simulink model "Bossi_Emanuele_EE460S3D_R99"  (R2025a)
settings: Solver=FixedStepDiscrete  StartTime=0.0  StopTime=120  FixedStep=dt0  RelTol=1e-3  EnableMultiTasking=on
PostLoadFcn:
  | %Set the size for the model
  | set_param(gcs,'Location',[10 10 1270 970])
  | %Set the zoom factor for the model
  | set_param(gcs,'ZoomFactor','100')
InitFcn:
  | tic
  | Bossi_Emanuele_EE460_Final
  | INIT_S3D_01
StartFcn:
  | tend0=toc;
  | tic;
StopFcn:
  | tend=toc;
  | disp(['Simulation time = ' num2str(tout(end)) ' sec'])
  | disp(['Real time = ' num2str(tend) ' sec'])
  | title('DONE')
  | SCORE=round((max(0,120-tout(end)-tend0))*4+10*(40-FuelBurned)+sum(100*double(PDONE)-100*double(PDONE<.5)));
  | PlotS3D(PlotInput);
  | text(15,22,['S: ' num2str(SCORE)]);
  | % Reset color scheme back to normal defaults
  | figure()
  | blkwhitebg('w');
  | close
values from neighbouring files (symbols this model uses):
  A_obs = [ 0  1  0  0  0  0 ... (first row only)    [Bossi_Emanuele_EE460_Final.m]
  B_obs = [ 0     0     0 ... (first row only)    [Bossi_Emanuele_EE460_Final.m]
  C_obs = [ 1 0 0 0 0 0 ... (first row only)    [Bossi_Emanuele_EE460_Final.m]
  d2r = pi/180    (= 0.0174532925199)    [INIT_S3D_01.m]
  D_obs = [ 0     0     0 ... (first row only)    [Bossi_Emanuele_EE460_Final.m]
  dt = 0.01    [INIT_S3D_01.m]
  dt0 = 0.001    [INIT_S3D_01.m]
  fr = 100    [INIT_S3D_01.m]
  G = [1,  1, -1, -1,  0,  0,  0,  0 ... (first row only)    [Bossi_Emanuele_EE460_Final.m]
  G_obs = eye(6)    [Bossi_Emanuele_EE460_Final.m]
  HM_S = 250    [INIT_S3D_01.m]
  HM_U = 500    [INIT_S3D_01.m]
  J = Jbase+JC0+JF+M*(Xcg^2+Ycg^2)    [INIT_S3D_01.m]
  Jbase = JC1+4*Ja+2*Ma*da^2+2*Ma*db^2    [INIT_S3D_01.m]
  JC0 = MC0/2    (= 10.2101761242)    [INIT_S3D_01.m]
  Kdtheta = 2 * zeta_th * wn_th * J_eff    [Bossi_Emanuele_EE460_Final.m]
  Kdtheta_fail = 2 * zeta_th_fail * wn_th_fail * J_eff    [Bossi_Emanuele_EE460_Final.m]
  Kdx = 2 * zeta_xy * wn_xy * M_eff    [Bossi_Emanuele_EE460_Final.m]
  Kdx_fail = 2 * zeta_xy_fail * wn_xy_fail * M_eff    [Bossi_Emanuele_EE460_Final.m]
  Kdy = 2 * zeta_xy * wn_xy * M_eff    [Bossi_Emanuele_EE460_Final.m]
  Kdy_fail = 2 * zeta_xy_fail * wn_xy_fail * M_eff    [Bossi_Emanuele_EE460_Final.m]
  Kptheta = J_eff * wn_th^2    [Bossi_Emanuele_EE460_Final.m]
  Kptheta_fail = J_eff * wn_th_fail^2    [Bossi_Emanuele_EE460_Final.m]
  Kpx = M_eff * wn_xy^2    [Bossi_Emanuele_EE460_Final.m]
  Kpx_fail = M_eff * wn_xy_fail^2    [Bossi_Emanuele_EE460_Final.m]
  Kpy = M_eff * wn_xy^2    [Bossi_Emanuele_EE460_Final.m]
  Kpy_fail = M_eff * wn_xy_fail^2    [Bossi_Emanuele_EE460_Final.m]
  L13 = sqrt(10)    [INIT_S3D_01.m]
  L24 = sqrt(6.25)    [INIT_S3D_01.m]
  LVL = LVL12    [INIT_S3D_01.m]
  M = MC+M1+M2+M3+M4+4*Ma    [INIT_S3D_01.m]
  M1 = LVL.M1    [INIT_S3D_01.m]
  M2 = LVL.M2    [INIT_S3D_01.m]
  M3 = LVL.M3    [INIT_S3D_01.m]
  M4 = LVL.M4    [INIT_S3D_01.m]
  max_qddot = [max_qddot_x; max_qddot_y; max_qddot_theta]    [Bossi_Emanuele_EE460_Final.m]
  mdti = (1/300)    (= 0.00333333333333)    [INIT_S3D_01.m]
  P = [1  1 -1 -1  0  0  0  0 ... (first row only)    [Bossi_Emanuele_EE460_Final.m]
  Pdata = [LVL.P1 LVL.P2 LVL.P3 LVL.P4]    [INIT_S3D_01.m]    (also in PlotS3D.m = R*[xt1;yt1+[0 3*tt*TV(idx-13)*TSIG(idx-13) 0]])
  PTvec = [Pdata(:,1);Pdata(:,2);Pdata(:,3);Pdata(:,4) ... (first row only)    [INIT_S3D_01.m]
  Q_obs = eye(6)    [Bossi_Emanuele_EE460_Final.m]
  r2d = 180/pi    (= 57.2957795131)    [INIT_S3D_01.m]
  r_bang = 0.5    [Bossi_Emanuele_EE460_Final.m]
  Sconfig = 1    [Bossi_Emanuele_EE460_Final.m]
  SLIM = [-100 100 ... (first row only)    [INIT_S3D_01.m]
  SQ = [.005 .01 .004 .005 .01 .004 .02 .01 .4]'    [INIT_S3D_01.m]
  SSF = 1./SQ    [INIT_S3D_01.m]
  tau = 0.5    [Bossi_Emanuele_EE460_Final.m]
  TOLdata = [LVL.P1tol LVL.P2tol LVL.P3tol LVL.P4tol]    [INIT_S3D_01.m]
  ULIM = [[Umin Umax];0 0;0 0]    [INIT_S3D_01.m]
undefined symbols (not defined in the file or in its folder): den_lp, den_lp2, DiscIntNeverNeededParam, dt1_bang_3, dt2_bang_3, dtc_bang_3, num_lp, num_lp2, q0_1
libraries: simulink x87, matrix_library x4, sl3dlib x1, aerolibutil x1, aerolibanimutils x1
(part 2 of 8)

== system Bossi_Emanuele_EE460S3D_R99/ControlLaw/ControlAllocation/A ==
  Y_IN : Inport
  Bus Creator : BusCreator  Inputs=2
  Bus Selector : BusSelector  OutputSignals=PT,Minv
  Constant1 : Constant  Value=P
  Constant2 : Constant  Value=P
  Gain : Gain  Gain=2
  Invert 3x3 Matrix : aerolibutil/Invert  3x3 Matrix
  MatrixMultiply{,1..3} (4 alike) : Product  Multiplication=Matrix(*)
  Transpose : Math  Operator=transpose
  WTI : Subsystem
  Out1 : Outport
  wires:
  Y_IN/1 -> WTI/1(Y_IN)
  WTI/1(Out1) -> MatrixMultiply3/1, MatrixMultiply1/2
  Constant1/1 -> MatrixMultiply1/1
  MatrixMultiply1/1 -> MatrixMultiply2/1
  Constant2/1 -> Transpose/1
  Transpose/1 -> Bus Creator/2, MatrixMultiply2/2  "PT"
  MatrixMultiply2/1 -> Invert 3x3 Matrix/1  "M"
  MatrixMultiply/1 -> MatrixMultiply3/2
  MatrixMultiply3/1 -> Gain/1  "A"
  Gain/1 -> Out1/1  "2A"
  Invert 3x3 Matrix/1 -> Bus Creator/1  "Minv"
  Bus Creator/1 -> Bus Selector/1
  Bus Selector/1 -> MatrixMultiply/1  "<PT>"
  Bus Selector/2 -> MatrixMultiply/2  "<Minv>"

== system Bossi_Emanuele_EE460S3D_R99/ControlLaw/ControlAllocation/BodyAxisModeling ==
  uP_cmd : Inport  PortDimensions=3
  theta_rad : Inport  Port=2
  Bus Creator : BusCreator  Inputs=5
  Bus Creator1 : BusCreator  Inputs=4
  Bus Selector : BusSelector  OutputSignals=Fx_N,c,c,Fy_N,Fy_N,s,Fx_N,s,Mz_Nm
  Bus Selector1 : BusSelector  OutputSignals=cFx,sFy,cFy,sFx
  Demux1 : Demux  Outputs=3
  FxB_sum1 : Sum  Inputs=|++
  Mux2 : Mux  Inputs=3
  Sum1 : Sum
  cFx1 : Product
  cFy1 : Product
  cos_theta1 : Trigonometry  Operator=cos
  neg2 : Gain  Gain=-1
  sFx1 : Product
  sFy1 : Product
  sin_theta1 : Trigonometry
  Out1 : Outport
  wires:
  uP_cmd/1 -> Demux1/1  "uP_cmd"
  cos_theta1/1 -> Bus Creator/1  "c"
  sin_theta1/1 -> Bus Creator/2  "s"
  Demux1/1 -> Bus Creator/3  "Fx_N"
  Demux1/2 -> Bus Creator/4  "Fy_N"
  Demux1/3 -> Bus Creator/5  "Mz_Nm"
  Bus Creator/1 -> Bus Selector/1
  Bus Selector/1 -> cFx1/1  "<Fx_N>"
  Bus Selector/2 -> cFx1/2  "<c>"
  Bus Selector/3 -> cFy1/1  "<c>"
  Bus Selector/4 -> cFy1/2  "<Fy_N>"
  Bus Selector/5 -> sFy1/1  "<Fy_N>"
  Bus Selector/6 -> sFy1/2  "<s>"
  Bus Selector/7 -> sFx1/1  "<Fx_N>"
  Bus Selector/8 -> sFx1/2  "<s>"
  cFx1/1 -> Bus Creator1/1  "cFx"
  cFy1/1 -> Bus Creator1/2  "cFy"
  sFy1/1 -> Bus Creator1/3  "sFy"
  sFx1/1 -> Bus Creator1/4  "sFx"
  Bus Creator1/1 -> Bus Selector1/1
  neg2/1 -> Sum1/2
  Bus Selector/9 -> Mux2/3  "<Mz_Nm>"
  Bus Selector1/1 -> FxB_sum1/1  "<cFx>"
  Bus Selector1/2 -> FxB_sum1/2  "<sFy>"
  FxB_sum1/1 -> Mux2/1  "FxB_pos"
  Bus Selector1/3 -> Sum1/1  "<cFy>"
  Bus Selector1/4 -> neg2/1  "<sFx>"
  Sum1/1 -> Mux2/2  "FyB_pos"
  theta_rad/1 -> sin_theta1/1, cos_theta1/1
  Mux2/1 -> Out1/1  "uP_body"

== system Bossi_Emanuele_EE460S3D_R99/ControlLaw/ControlAllocation/R_theta ==
  In2 : Inport
  Bus Creator : BusCreator  Inputs=5
  Bus Selector : BusSelector  OutputSignals=c,minus_s,z0,s,c,z0,z0,z0,z1
  Constant : Constant  Value=0  SampleTime=dt
  Constant1 : Constant  SampleTime=dt
  Cos : Trigonometry  Operator=cos
  Gain : Gain  Gain=-1
  Matrix Concatenate : Concatenate  NumInputs=3  Mode=Multidimensional array
  Mux : Mux  Inputs=3
  Mux1 : Mux  Inputs=3
  Mux2 : Mux  Inputs=3
  Reshape : Reshape  OutputDimensionality=Customize  OutputDimensions=[1,3]
  Reshape1 : Reshape  OutputDimensionality=Customize  OutputDimensions=[1,3]
  Reshape2 : Reshape  OutputDimensionality=Customize  OutputDimensions=[1,3]
  Sin : Trigonometry
  Out1 : Outport
  wires:
  In2/1 -> Sin/1, Cos/1
  Sin/1 -> Gain/1, Bus Creator/4  "s"
  Cos/1 -> Bus Creator/3  "c"
  Gain/1 -> Bus Creator/5  "minus_s"
  Constant/1 -> Bus Creator/1  "z0"
  Constant1/1 -> Bus Creator/2  "z1"
  Bus Creator/1 -> Bus Selector/1
  Matrix Concatenate/1 -> Out1/1  "R"
  Bus Selector/1 -> Mux/1  "<c>"
  Bus Selector/2 -> Mux/2  "<minus_s>"
  Bus Selector/3 -> Mux/3  "<z0>"
  Bus Selector/4 -> Mux1/1  "<s>"
  Bus Selector/5 -> Mux1/2  "<c>"
  Bus Selector/6 -> Mux1/3  "<z0>"
  Bus Selector/7 -> Mux2/1  "<z0>"
  Bus Selector/8 -> Mux2/2  "<z0>"
  Bus Selector/9 -> Mux2/3  "<z1>"
  Mux/1 -> Reshape/1
  Reshape/1 -> Matrix Concatenate/1
  Reshape1/1 -> Matrix Concatenate/2
  Mux1/1 -> Reshape1/1
  Mux2/1 -> Reshape2/1
  Reshape2/1 -> Matrix Concatenate/3

== system Bossi_Emanuele_EE460S3D_R99/ControlLaw/ControlAllocation/ThrusterFailure ==
  Y_IN : Inport
  Bus Creator1 : BusCreator  Inputs=8
  Bus Creator2 : BusCreator  Inputs=8
  Bus Selector3 : BusSelector  OutputSignals=U1fail,U2fail,U3fail,U4fail,U5fail,U6fail,U7fail,U8fail
  Bus Selector4 : BusSelector  OutputSignals=U1est,U2est,U3est,U4est,U5est,U6est,U7est,U8est
  Bus to Vector : BusToVector
  Bus to Vector1 : BusToVector
  Constant : Constant  Value=P
  Data Type Conversion : DataTypeConversion  OutDataTypeStr=double  SaturateOnIntegerOverflow=off  RndMeth=Floor
  Data Type Conversion1 : DataTypeConversion  OutDataTypeStr=double  SaturateOnIntegerOverflow=off  RndMeth=Floor
  MatrixMultiply : Product  Multiplication=Matrix(*)
  MatrixMultiply1 : Product
  Out1 : Outport
  Out2 : Outport  Port=2
  wires:
  Bus Selector3/5 -> Bus Creator1/5  "<U5fail>"
  Data Type Conversion1/1 -> MatrixMultiply1/2
  Bus Selector3/3 -> Bus Creator1/3  "<U3fail>"
  Bus Selector4/6 -> Bus Creator2/6  "<U6est>"
  Bus Selector4/4 -> Bus Creator2/4  "<U4est>"
  Bus Selector3/4 -> Bus Creator1/4  "<U4fail>"
  Bus Selector4/2 -> Bus Creator2/2  "<U2est>"
  Bus Selector3/2 -> Bus Creator1/2  "<U2fail>"
  Bus Selector3/7 -> Bus Creator1/7  "<U7fail>"
  Bus to Vector/1 -> Data Type Conversion/1
  Bus Creator2/1 -> Bus to Vector1/1
  Bus Creator1/1 -> Bus to Vector/1
  Bus Selector3/8 -> Bus Creator1/8  "<U8fail>"
  Bus Selector4/8 -> Bus Creator2/8  "<U8est>"
  Bus Selector4/3 -> Bus Creator2/3  "<U3est>"
  Bus to Vector1/1 -> Data Type Conversion1/1
  Data Type Conversion/1 -> MatrixMultiply1/1
  Bus Selector3/1 -> Bus Creator1/1  "<U1fail>"
  Bus Selector4/1 -> Bus Creator2/1  "<U1est>"
  Bus Selector4/5 -> Bus Creator2/5  "<U5est>"
  Bus Selector4/7 -> Bus Creator2/7  "<U7est>"
  Bus Selector3/6 -> Bus Creator1/6  "<U6fail>"
  Y_IN/1 -> Bus Selector4/1, Bus Selector3/1
  MatrixMultiply1/1 -> Out2/1, MatrixMultiply/2  "Ufail_mod"
  Constant/1 -> MatrixMultiply/1
  MatrixMultiply/1 -> Out1/1  "Failures"

== system Bossi_Emanuele_EE460S3D_R99/ControlLaw/InputDataConditioning/Sconfig1 ==
  Sensors : Inport  PortDimensions=9
  xhat_2 : Inport  Port=2
  SensorFailures : Inport  Port=3
  Bus Creator : BusCreator  Inputs=9
  Bus Creator1 : BusCreator  Inputs=19
  Bus Selector : BusSelector  OutputSignals=x_m,xdot_mps,xddot_mps2,y_m,ydot_mps,yddot_mps2,theta_deg,thetadot_degps,thetaddot_degps2
  Bus Selector1 : BusSelector  OutputSignals=x_m,Fail_flags.S1fail,Xpos_m,xdot_mps,Fail_flags.S2fail,Xvel_mps,xddot_mps2,Fail_flags.S3fail,Xacc_mps2,y_m,Fail_flags.S4fail,Ypos_m,ydot_mps,Fail_flags.S5fail,Yvel_mps,yddot_mps2,Fail_flags.S6fail,Yacc_mps2,theta_deg,Fail_flags.S7fail,theta_pos_deg,thetadot_degps,Fail_flags.S8fail,theta_vel_degps,thetaddot_degps2,Fail_flags.S9fail,theta_acc_degreeps2
  Discrete Transfer Fcn{,1,3..4,6..7} (6 alike) : DiscreteTransferFcn  Numerator=num_lp  Denominator=den_lp
  Discrete Transfer Fcn{9..14} (6 alike) : DiscreteTransferFcn  Numerator=num_lp2  Denominator=den_lp2
  SensedValues : Subsystem
  Sum{,1..5} (6 alike) : Sum  Inputs=|++
  Switch{,1..8} (9 alike) : Switch  Criteria=u2 > Threshold  SaturateOnIntegerOverflow=off  InputSameDT=off
  Y_IN : Outport
  wires:
  Bus Creator/1 -> Y_IN/1  "SensorGain"
  Discrete Transfer Fcn/1 -> Sum/1
  Discrete Transfer Fcn9/1 -> Sum/2
  Discrete Transfer Fcn1/1 -> Sum1/1
  Discrete Transfer Fcn10/1 -> Sum1/2
  Discrete Transfer Fcn3/1 -> Sum2/1
  Sum/1 -> Bus Creator/1  "Xpos_m"
  Sum1/1 -> Bus Creator/2  "Xvel_mps"
  Discrete Transfer Fcn4/1 -> Sum3/1
  Sum3/1 -> Bus Creator/5  "Yvel_mps"
  Sum2/1 -> Bus Creator/4  "Ypos_m"
  Discrete Transfer Fcn6/1 -> Sum4/1
  Sum4/1 -> Bus Creator/7  "theta_pos_deg"
  Discrete Transfer Fcn7/1 -> Sum5/1
  Sum5/1 -> Bus Creator/8  "theta_vel_degps"
  Discrete Transfer Fcn11/1 -> Sum2/2
  Discrete Transfer Fcn12/1 -> Sum3/2
  Discrete Transfer Fcn13/1 -> Sum4/2
  Discrete Transfer Fcn14/1 -> Sum5/2
  Sensors/1 -> SensedValues/1(Sensors)  "Sensors"
  xhat_2/1 -> Bus Selector/1  "xhat"
  SensedValues/1(Out1) -> Bus Creator1/1
  SensedValues/2(Out2) -> Bus Creator1/2
  SensedValues/3(Out3) -> Bus Creator1/3
  SensedValues/4(Out4) -> Bus Creator1/4
  SensedValues/5(Out5) -> Bus Creator1/5
  SensedValues/6(Out6) -> Bus Creator1/6
  SensedValues/7(Out7) -> Bus Creator1/7
  SensedValues/8(Out8) -> Bus Creator1/8
  SensedValues/9(Out9) -> Bus Creator1/9
  SensorFailures/1 -> Bus Creator1/10  "Fail_flags"
  Bus Selector/1 -> Bus Creator1/11  "<x_m>"
  Bus Selector/2 -> Bus Creator1/12  "<xdot_mps>"
  Bus Selector/3 -> Bus Creator1/13  "<xddot_mps2>"
  Bus Selector/4 -> Bus Creator1/14  "<y_m>"
  Bus Selector/5 -> Bus Creator1/15  "<ydot_mps>"
  Bus Selector/6 -> Bus Creator1/16  "<yddot_mps2>"
  Bus Selector/7 -> Bus Creator1/17  "<theta_deg>"
  Bus Selector/8 -> Bus Creator1/18  "<thetadot_degps>"
  Bus Selector/9 -> Bus Creator1/19  "<thetaddot_degps2>"
  Bus Creator1/1 -> Bus Selector1/1
  Bus Selector1/1 -> Switch/1  "<x_m>"
  Bus Selector1/2 -> Switch/2  "<S1fail>"
  Bus Selector1/3 -> Switch/3  "<Xpos_m>"
  Switch/1 -> Discrete Transfer Fcn/1
  Bus Selector1/4 -> Switch1/1  "<xdot_mps>"
  Bus Selector1/5 -> Switch1/2  "<S2fail>"
  Bus Selector1/6 -> Switch1/3  "<Xvel_mps>"
  Bus Selector1/7 -> Switch2/1  "<xddot_mps2>"
  Bus Selector1/8 -> Switch2/2  "<S3fail>"
  Bus Selector1/9 -> Switch2/3  "<Xacc_mps2>"
  Bus Selector1/11 -> Switch3/2  "<S4fail>"
  Bus Selector1/12 -> Switch3/3  "<Ypos_m>"
  Bus Selector1/10 -> Switch3/1  "<y_m>"
  Bus Selector1/13 -> Switch4/1  "<ydot_mps>"
  Bus Selector1/14 -> Switch4/2  "<S5fail>"
  Bus Selector1/15 -> Switch4/3  "<Yvel_mps>"
  Bus Selector1/16 -> Switch5/1  "<yddot_mps2>"
  Bus Selector1/17 -> Switch5/2  "<S6fail>"
  Bus Selector1/18 -> Switch5/3  "<Yacc_mps2>"
  Bus Selector1/20 -> Switch6/2  "<S7fail>"
  Bus Selector1/21 -> Switch6/3  "<theta_pos_deg>"
  Bus Selector1/19 -> Switch6/1  "<theta_deg>"
  Bus Selector1/24 -> Switch7/3  "<theta_vel_degps>"
  Bus Selector1/23 -> Switch7/2  "<S8fail>"
  Bus Selector1/22 -> Switch7/1  "<thetadot_degps>"
  Bus Selector1/27 -> Switch8/3  "<theta_acc_degreeps2>"
  Bus Selector1/26 -> Switch8/2  "<S9fail>"
  Bus Selector1/25 -> Switch8/1  "<thetaddot_degps2>"
  Switch1/1 -> Discrete Transfer Fcn9/1, Discrete Transfer Fcn1/1
  Switch2/1 -> Bus Creator/3, Discrete Transfer Fcn10/1  "Xacc_mps2"
  Switch4/1 -> Discrete Transfer Fcn11/1, Discrete Transfer Fcn4/1
  Switch3/1 -> Discrete Transfer Fcn3/1
  Switch5/1 -> Bus Creator/6, Discrete Transfer Fcn12/1  "Yacc_mps2"
  Switch8/1 -> Bus Creator/9, Discrete Transfer Fcn14/1  "theta_acc_degreeps2"
  Switch7/1 -> Discrete Transfer Fcn13/1, Discrete Transfer Fcn7/1
  Switch6/1 -> Discrete Transfer Fcn6/1

== system Bossi_Emanuele_EE460S3D_R99/ControlLaw/Observer/InternalObserver ==
  CAout : Inport
  Y_IN : Inport  Port=2
  ABM_INT : Subsystem
  Bus Creator : BusCreator  Inputs=2
  Bus Selector : BusSelector  OutputSignals=Xpos_m,Xvel_mps,Xacc_mps2,Ypos_m,Yvel_mps,Yacc_mps2,theta_pos_deg,theta_vel_degps,theta_acc_degreeps2
  Bus Selector1 : BusSelector  OutputSignals=Y_IN,X_hat
  C_obs : Subsystem
  Gain1 : Gain  Gain=A_obs  Multiplication=Matrix(K*u)
  Gain3 : Gain  Gain=D_obs  Multiplication=Matrix(K*u)
  Gain4 : Gain  Gain=B_obs  Multiplication=Matrix(K*u)
  L : Subsystem
  MatrixMultiply : Product  Multiplication=Matrix(*)
  MatrixMultiply1 : Product  Multiplication=Matrix(*)
  Mux : Mux  Inputs=9
  Sum : Sum  Inputs=|-+
  Sum1 : Sum  Inputs=|++
  Sum2 : Sum  Inputs=|++
  Sum3 : Sum  Inputs=++|
  Unit Delay : UnitDelay  SampleTime=dt  HasFrameUpgradeWarning=on
  xdot_hat : Outport
  x_hat : Outport  Port=2
  wires:
  MatrixMultiply/1 -> Sum2/1
  Sum2/1 -> Sum1/2
  Sum1/1 -> Unit Delay/1, ABM_INT/1(DX)  "Xdot_hat"
  Gain1/1 -> Sum2/2
  Gain3/1 -> Sum3/1
  Sum3/1 -> Sum/1  "y_hat"
  Gain4/1 -> Sum1/1
  ABM_INT/1(X) -> x_hat/1, Gain1/1, Bus Creator/1  "X_hat"
  Y_IN/1 -> Bus Selector/1, L/3(In1), L/2(Y_IN1), L/1(Y_IN), Bus Creator/2
  Mux/1 -> Sum/2
  Bus Selector/1 -> Mux/1  "<Xpos_m>"
  Bus Selector/2 -> Mux/2  "<Xvel_mps>"
  Bus Selector/3 -> Mux/3  "<Xacc_mps2>"
  Bus Selector/4 -> Mux/4  "<Ypos_m>"
  Bus Selector/5 -> Mux/5  "<Yvel_mps>"
  Bus Selector/6 -> Mux/6  "<Yacc_mps2>"
  Bus Selector/7 -> Mux/7  "<theta_pos_deg>"
  Bus Selector/8 -> Mux/8  "<theta_vel_degps>"
  Bus Selector/9 -> Mux/9  "<theta_acc_degreeps2>"
  L/1(Out1) -> MatrixMultiply/1
  Sum/1 -> MatrixMultiply/2
  C_obs/1(Out1) -> MatrixMultiply1/1
  Bus Creator/1 -> Bus Selector1/1
  MatrixMultiply1/1 -> Sum3/2
  Bus Selector1/1 -> C_obs/1(Y_IN)  "<Y_IN>"
  Bus Selector1/2 -> MatrixMultiply1/2  "<X_hat>"
  CAout/1 -> Gain3/1, Gain4/1
  Unit Delay/1 -> xdot_hat/1  "Xdot_hat"

== system Bossi_Emanuele_EE460S3D_R99/ControlLaw/Observer/SensorFailureHandling ==
  CAout : Inport
  Y_IN : Inport  Port=2
  Bus Creator : BusCreator  Inputs=3
  Bus Creator1 : BusCreator  Inputs=21
  Bus Creator2 : BusCreator  Inputs=9
  Bus Creator5 : BusCreator  Inputs=18
  Bus Selector : BusSelector  OutputSignals=Xpos_m,Xvel_mps,Xacc_mps2,Ypos_m,Yvel_mps,Yacc_mps2,theta_pos_deg,theta_vel_degps,theta_acc_degreeps2,S1fail,S2fail,S3fail,S4fail,S5fail,S6fail,S7fail,S8fail,S9fail
  Bus Selector1 : BusSelector  OutputSignals=Fx,Fy,Mz
  Bus Selector2 : BusSelector  OutputSignals=Fx,S3fail,Xacc_mps2,S2fail,Xvel_mps,S1fail,Xpos_m
  Bus Selector3 : BusSelector  OutputSignals=Fy,S6fail,Yacc_mps2,S5fail,Yvel_mps,S4fail,Ypos_m
  Bus Selector4 : BusSelector  OutputSignals=Mz,S9fail,theta_acc_degreeps2,S8fail,theta_vel_degps,S7fail,theta_pos_deg
  Bus Selector5 : BusSelector  OutputSignals=S1fail,S2fail,S3fail,S4fail,S5fail,S6fail,S7fail,S8fail,S9fail
  Bus Selector6 : BusSelector  OutputSignals=Xpos_m,Xvel_mps,Xacc_mps2,Ypos_m,Yvel_mps,Yacc_mps2,theta_pos_deg,theta_vel_degps,theta_acc_degreeps2
  Selector : Selector  InputPortWidth=3  IndexOptions=Index vector (dialog)  Indices=[1]  OutputSizes=1
  Selector1 : Selector  InputPortWidth=3  IndexOptions=Index vector (dialog)  Indices=[2]  OutputSizes=1
  Selector2 : Selector  InputPortWidth=3  IndexOptions=Index vector (dialog)  Indices=[3]  OutputSizes=1
  Theta : Subsystem
  X : Subsystem
  Y : Subsystem
  Out1 : Outport
  Out2 : Outport  Port=2
  wires:
  CAout/1 -> Out1/1, Selector2/1, Selector1/1, Selector/1
  Y_IN/1 -> Bus Selector5/1, Bus Selector/1
  Selector/1 -> Bus Creator/1  "Fx"
  Selector1/1 -> Bus Creator/2  "Fy"
  Selector2/1 -> Bus Creator/3  "Mz"
  Bus Creator/1 -> Bus Selector1/1
  Bus Selector/18 -> Bus Creator1/21  "<S9fail>"
  Bus Selector/17 -> Bus Creator1/20  "<S8fail>"
  Bus Selector/16 -> Bus Creator1/19  "<S7fail>"
  Bus Selector/15 -> Bus Creator1/18  "<S6fail>"
  Bus Selector/14 -> Bus Creator1/17  "<S5fail>"
  Bus Selector/13 -> Bus Creator1/16  "<S4fail>"
  Bus Selector/12 -> Bus Creator1/15  "<S3fail>"
  Bus Selector/11 -> Bus Creator1/14  "<S2fail>"
  Bus Selector/10 -> Bus Creator1/13  "<S1fail>"
  Bus Selector/9 -> Bus Creator1/12  "<theta_acc_degreeps2>"
  Bus Selector/8 -> Bus Creator1/11  "<theta_vel_degps>"
  Bus Selector/7 -> Bus Creator1/10  "<theta_pos_deg>"
  Bus Selector/6 -> Bus Creator1/9  "<Yacc_mps2>"
  Bus Selector/5 -> Bus Creator1/8  "<Yvel_mps>"
  Bus Selector/4 -> Bus Creator1/7  "<Ypos_m>"
  Bus Selector/3 -> Bus Creator1/6  "<Xacc_mps2>"
  Bus Selector/2 -> Bus Creator1/5  "<Xvel_mps>"
  Bus Selector/1 -> Bus Creator1/4  "<Xpos_m>"
  Bus Selector1/3 -> Bus Creator1/3  "<Mz>"
  Bus Selector1/2 -> Bus Creator1/2  "<Fy>"
  Bus Selector1/1 -> Bus Creator1/1  "<Fx>"
  Bus Creator1/1 -> Bus Selector3/1, Bus Selector4/1, Bus Selector2/1
  Bus Creator5/1 -> Out2/1  "Y_IN"
  Bus Selector2/1 -> X/1(In1)  "<Fx>"
  Bus Selector2/2 -> X/2(In2)  "<S3fail>"
  Bus Selector2/3 -> X/3(In3)  "<Xacc_mps2>"
  Bus Selector2/4 -> X/4(In4)  "<S2fail>"
  Bus Selector2/5 -> X/5(In5)  "<Xvel_mps>"
  Bus Selector2/6 -> X/6(In6)  "<S1fail>"
  Bus Selector2/7 -> X/7(In7)  "<Xpos_m>"
  Bus Selector3/1 -> Y/1(In1)  "<Fy>"
  Bus Selector3/2 -> Y/2(In2)  "<S6fail>"
  Bus Selector3/3 -> Y/3(In3)  "<Yacc_mps2>"
  Bus Selector3/4 -> Y/4(In4)  "<S5fail>"
  Bus Selector3/5 -> Y/5(In5)  "<Yvel_mps>"
  Bus Selector3/6 -> Y/6(In6)  "<S4fail>"
  Bus Selector3/7 -> Y/7(In7)  "<Ypos_m>"
  Bus Selector4/1 -> Theta/1(In1)  "<Mz>"
  Bus Selector4/2 -> Theta/2(In2)  "<S9fail>"
  Bus Selector4/3 -> Theta/3(In3)  "<theta_acc_degreeps2>"
  Bus Selector4/4 -> Theta/4(In4)  "<S8fail>"
  Bus Selector4/5 -> Theta/5(In5)  "<theta_vel_degps>"
  Bus Selector4/6 -> Theta/6(In6)  "<S7fail>"
  Bus Selector4/7 -> Theta/7(In7)  "<theta_pos_deg>"
  X/1(Out1) -> Bus Creator2/1
  X/2(Out2) -> Bus Creator2/2
  X/3(Out3) -> Bus Creator2/3
  Y/1(Out1) -> Bus Creator2/4
  Y/2(Out2) -> Bus Creator2/5
  Y/3(Out3) -> Bus Creator2/6
  Theta/1(Out1) -> Bus Creator2/7
  Theta/2(Out2) -> Bus Creator2/8
  Theta/3(Out3) -> Bus Creator2/9
  Bus Creator2/1 -> Bus Selector6/1
  Bus Selector6/1 -> Bus Creator5/1  "<Xpos_m>"
  Bus Selector6/2 -> Bus Creator5/2  "<Xvel_mps>"
  Bus Selector6/3 -> Bus Creator5/3  "<Xacc_mps2>"
  Bus Selector6/4 -> Bus Creator5/4  "<Ypos_m>"
  Bus Selector6/5 -> Bus Creator5/5  "<Yvel_mps>"
  Bus Selector6/6 -> Bus Creator5/6  "<Yacc_mps2>"
  Bus Selector6/7 -> Bus Creator5/7  "<theta_pos_deg>"
  Bus Selector6/8 -> Bus Creator5/8  "<theta_vel_degps>"
  Bus Selector6/9 -> Bus Creator5/9  "<theta_acc_degreeps2>"
  Bus Selector5/1 -> Bus Creator5/10  "<S1fail>"
  Bus Selector5/2 -> Bus Creator5/11  "<S2fail>"
  Bus Selector5/3 -> Bus Creator5/12  "<S3fail>"
  Bus Selector5/4 -> Bus Creator5/13  "<S4fail>"
  Bus Selector5/5 -> Bus Creator5/14  "<S5fail>"
  Bus Selector5/6 -> Bus Creator5/15  "<S6fail>"
  Bus Selector5/7 -> Bus Creator5/16  "<S7fail>"
  Bus Selector5/8 -> Bus Creator5/17  "<S8fail>"
  Bus Selector5/9 -> Bus Creator5/18  "<S9fail>"

== system Bossi_Emanuele_EE460S3D_R99/ControlLaw/Regulator/NoFailures ==
  In1 : Inport
  Action Port : ActionPort  ActionPortLabel=if(u1 == 0)
  AngleWrapper : Subsystem
  Bus Selector1 : BusSelector  OutputSignals=x_cmd,x_m,xdot_mps,y_cmd,y_m,ydot_mps,theta_cmd,theta_deg,thetadot_degps
  Gain : Gain  Gain=Kpx
  Gain1 : Gain  Gain=Kdx
  Gain2 : Gain  Gain=Kpy
  Gain3 : Gain  Gain=Kdy
  Gain4 : Gain  Gain=Kptheta
  Gain5 : Gain  Gain=Kdtheta
  Mux : Mux  Inputs=3
  Scope : Scope  NumInputPorts=2
      settings: ActiveDisplayYMinimum=-25.943403384100005  ActiveDisplayYMaximum=26.147870706177621  DataLoggingVariableName=ScopeData3
  Scope1 : Scope  NumInputPorts=2
      settings: ActiveDisplayYMinimum=-4.47505390682404  ActiveDisplayYMaximum=19.513493144834005  DataLoggingVariableName=ScopeData5
  Scope2 : Scope  NumInputPorts=2
      settings: ActiveDisplayYMinimum=-6.9525163364863216  ActiveDisplayYMaximum=8.7180069928828718  DataLoggingVariableName=ScopeData6
  Sum : Sum  Inputs=|+-
  Sum2 : Sum  Inputs=+-
  Sum3 : Sum  Inputs=|+-
  Sum5 : Sum  Inputs=+-
  Sum6 : Sum  Inputs=|+-
  Sum8 : Sum  Inputs=+-
  uP_cmd : Outport
  wires:
  Sum2/1 -> Mux/1  "Fx"
  Bus Selector1/4 -> Scope1/1, Sum3/1  "<y_cmd>"
  Gain2/1 -> Sum5/1
  Gain4/1 -> Sum8/1
  AngleWrapper/1(Out1) -> Gain4/1
  Bus Selector1/2 -> Scope/2, Sum/2  "<x_m>"
  Sum6/1 -> AngleWrapper/1(In1)  "theta_deg"
  Bus Selector1/7 -> Scope2/1, Sum6/1  "<theta_cmd>"
  Sum/1 -> Gain/1
  Gain3/1 -> Sum5/2
  Bus Selector1/1 -> Scope/1, Sum/1  "<x_cmd>"
  Sum8/1 -> Mux/3  "Mz"
  Bus Selector1/9 -> Gain5/1  "<thetadot_degps>"
  Sum5/1 -> Mux/2  "Fy"
  Bus Selector1/3 -> Gain1/1  "<xdot_mps>"
  Gain5/1 -> Sum8/2
  Gain1/1 -> Sum2/2
  Bus Selector1/5 -> Scope1/2, Sum3/2  "<y_m>"
  Sum3/1 -> Gain2/1
  Bus Selector1/8 -> Scope2/2, Sum6/2  "<theta_deg>"
  Gain/1 -> Sum2/1
  In1/1 -> Bus Selector1/1
  Mux/1 -> uP_cmd/1  "uP"
  Bus Selector1/6 -> Gain3/1  "<ydot_mps>"

== system Bossi_Emanuele_EE460S3D_R99/ControlLaw/Regulator/ThrusterFailures ==
  In1 : Inport
  Action Port : ActionPort  ActionPortLabel=else
  AngleWrapper : Subsystem
  Bus Selector1 : BusSelector  OutputSignals=x_cmd,x_m,xdot_mps,y_cmd,y_m,ydot_mps,theta_cmd,theta_deg,thetadot_degps
  Gain : Gain  Gain=Kpx_fail
  Gain1 : Gain  Gain=Kdx_fail
  Gain2 : Gain  Gain=Kpy_fail
  Gain3 : Gain  Gain=Kdy_fail
  Gain4 : Gain  Gain=Kptheta_fail
  Gain5 : Gain  Gain=Kdtheta_fail
  Mux : Mux  Inputs=3
  Scope : Scope  NumInputPorts=2
      settings: ActiveDisplayYMinimum=-29.197116643477266  ActiveDisplayYMaximum=28.687775741072066  DataLoggingVariableName=ScopeData3
  Scope1 : Scope  NumInputPorts=2
      settings: ActiveDisplayYMinimum=-4.47505390682404  ActiveDisplayYMaximum=19.513493144834005  DataLoggingVariableName=ScopeData5
  Scope2 : Scope  NumInputPorts=2
      settings: ActiveDisplayYMinimum=-6.9525163364863216  ActiveDisplayYMaximum=8.7180069928828718  DataLoggingVariableName=ScopeData6
  Sum : Sum  Inputs=|+-
  Sum2 : Sum  Inputs=+-
  Sum3 : Sum  Inputs=|+-
  Sum5 : Sum  Inputs=+-
  Sum6 : Sum  Inputs=|+-
  Sum8 : Sum  Inputs=+-
  uP_cmd : Outport
  wires:
  Sum2/1 -> Mux/1  "Fx"
  Bus Selector1/4 -> Scope1/1, Sum3/1  "<y_cmd>"
  Gain2/1 -> Sum5/1
  Gain4/1 -> Sum8/1
  AngleWrapper/1(Out1) -> Gain4/1
  Bus Selector1/2 -> Scope/2, Sum/2  "<x_m>"
  Sum6/1 -> AngleWrapper/1(In1)  "theta_deg"
  Bus Selector1/7 -> Scope2/1, Sum6/1  "<theta_cmd>"
  Sum/1 -> Gain/1
  Gain3/1 -> Sum5/2
  Bus Selector1/1 -> Scope/1, Sum/1  "<x_cmd>"
  Sum8/1 -> Mux/3  "Mz"
  Bus Selector1/9 -> Gain5/1  "<thetadot_degps>"
  Sum5/1 -> Mux/2  "Fy"
  Bus Selector1/3 -> Gain1/1  "<xdot_mps>"
  Gain5/1 -> Sum8/2
  Gain1/1 -> Sum2/2
  Bus Selector1/5 -> Scope1/2, Sum3/2  "<y_m>"
  Sum3/1 -> Gain2/1
  Bus Selector1/8 -> Scope2/2, Sum6/2  "<theta_deg>"
  Gain/1 -> Sum2/1
  In1/1 -> Bus Selector1/1
  Mux/1 -> uP_cmd/1  "uP"
  Bus Selector1/6 -> Gain3/1  "<ydot_mps>"

== system Bossi_Emanuele_EE460S3D_R99/S3D_Plant/Comm/P1 ==
  X : Inport
  Abs : Abs  SaturateOnIntegerOverflow=off
  Bus Selector2 : BusSelector  OutputSignals=x_m,y_m,tht_rad
  Compare To Constant : simulink/Logic and Bit Operations/Compare To Constant  relop=<=  const=1  OutDataTypeStr=boolean
  Compare To Constant1 : simulink/Logic and Bit Operations/Compare To Constant  relop=<=  const=TOLdata(3,Pdx)  OutDataTypeStr=boolean
  Compare To Constant2 : simulink/Logic and Bit Operations/Compare To Constant  relop=>=  const=LVL.Ptime(Pdx)/dt0  OutDataTypeStr=boolean
  Constant : Constant  Value=Pdata(1,Pdx)  SampleTime=dt0
  Constant1 : Constant  Value=Pdata(2,Pdx)  SampleTime=dt0
  Constant3 : Constant  Value=0  SampleTime=dt0
  Constant4 : Constant  SampleTime=dt0
  Constant7 : Constant  Value=Pdata(3,Pdx)  SampleTime=dt0
  DirectionCompensation2 : Subsystem
  Gain : Gain  Gain=1/(TOLdata(1,Pdx)^2)
  Gain1 : Gain  Gain=1/(TOLdata(2,Pdx)^2)
  Gain3 : Gain  Gain=d2r
  Gain4 : Gain  Gain=r2d
  Logical Operator : Logic  AllPortsSameDT=off  OutDataTypeStr=boolean
  Logical Operator1 : Logic  Operator=OR  AllPortsSameDT=off  OutDataTypeStr=boolean
  Product : Product
  Product1 : Product
  Sum : Sum  Inputs=|+-
  Sum1 : Sum  Inputs=|+-
  Sum3 : Sum  Inputs=|++
  Sum4 : Sum  Inputs=|+-
  Sum5 : Sum  Inputs=++|
  Switch : Switch  Criteria=u2 > Threshold  Threshold=.4  SaturateOnIntegerOverflow=off  InputSameDT=off
  Unit Delay1 : UnitDelay  SampleTime=dt0  HasFrameUpgradeWarning=on
  Unit Delay2 : UnitDelay  SampleTime=dt0  HasFrameUpgradeWarning=on
  COMM_OK : Outport
  COMM_DONE : Outport  Port=2
  wires:
  Gain4/1 -> Abs/1
  Sum4/1 -> DirectionCompensation2/1(In1)  "Delta_rad"
  Gain3/1 -> Sum4/2
  Constant7/1 -> Gain3/1
  Constant3/1 -> Switch/3
  Sum5/1 -> Switch/1
  Unit Delay1/1 -> Sum5/1
  Constant4/1 -> Sum5/2
  Logical Operator1/1 -> Unit Delay2/1, COMM_DONE/1
  Compare To Constant2/1 -> Logical Operator1/1
  Switch/1 -> Unit Delay1/1, Compare To Constant2/1
  Unit Delay2/1 -> Logical Operator1/2
  Sum3/1 -> Compare To Constant/1
  Compare To Constant/1 -> Logical Operator/1
  Abs/1 -> Compare To Constant1/1
  Product/1 -> Gain/1
  Compare To Constant1/1 -> Logical Operator/2
  Constant/1 -> Sum/2
  Logical Operator/1 -> Switch/2, COMM_OK/1
  Bus Selector2/1 -> Sum/1  "<x_m>"
  Bus Selector2/2 -> Sum1/1  "<y_m>"
  Constant1/1 -> Sum1/2
  X/1 -> Bus Selector2/1
  Sum1/1 -> Product1/1, Product1/2
  Gain/1 -> Sum3/1
  Sum/1 -> Product/1, Product/2
  Gain1/1 -> Sum3/2
  Bus Selector2/3 -> Sum4/1  "<tht_rad>"
  Product1/1 -> Gain1/1
  DirectionCompensation2/1(Out1) -> Gain4/1

== system Bossi_Emanuele_EE460S3D_R99/S3D_Plant/Comm/P2 ==
  X : Inport
  Abs : Abs  SaturateOnIntegerOverflow=off
  Bus Selector2 : BusSelector  OutputSignals=x_m,y_m,tht_rad
  Compare To Constant : simulink/Logic and Bit Operations/Compare To Constant  relop=<=  const=1  OutDataTypeStr=boolean
  Compare To Constant1 : simulink/Logic and Bit Operations/Compare To Constant  relop=<=  const=TOLdata(3,Pdx)  OutDataTypeStr=boolean
  Compare To Constant2 : simulink/Logic and Bit Operations/Compare To Constant  relop=>=  const=LVL.Ptime(Pdx)/dt0  OutDataTypeStr=boolean
  Constant : Constant  Value=Pdata(1,Pdx)  SampleTime=dt0
  Constant1 : Constant  Value=Pdata(2,Pdx)  SampleTime=dt0
  Constant3 : Constant  Value=0  SampleTime=dt0
  Constant4 : Constant  SampleTime=dt0
  Constant7 : Constant  Value=Pdata(3,Pdx)  SampleTime=dt0
  DirectionCompensation2 : Subsystem
  Gain : Gain  Gain=1/(TOLdata(1,Pdx)^2)
  Gain1 : Gain  Gain=1/(TOLdata(2,Pdx)^2)
  Gain3 : Gain  Gain=d2r
  Gain4 : Gain  Gain=r2d
  Logical Operator : Logic  AllPortsSameDT=off  OutDataTypeStr=boolean
  Logical Operator1 : Logic  Operator=OR  AllPortsSameDT=off  OutDataTypeStr=boolean
  Product : Product
  Product1 : Product
  Sum : Sum  Inputs=|+-
  Sum1 : Sum  Inputs=|+-
  Sum3 : Sum  Inputs=|++
  Sum4 : Sum  Inputs=|+-
  Sum5 : Sum  Inputs=++|
  Switch : Switch  Criteria=u2 > Threshold  Threshold=.4  SaturateOnIntegerOverflow=off  InputSameDT=off
  Unit Delay1 : UnitDelay  SampleTime=dt0  HasFrameUpgradeWarning=on
  Unit Delay2 : UnitDelay  SampleTime=dt0  HasFrameUpgradeWarning=on
  COMM_OK : Outport
  COMM_DONE : Outport  Port=2
  wires:
  Gain4/1 -> Abs/1
  DirectionCompensation2/1(Out1) -> Gain4/1
  Sum4/1 -> DirectionCompensation2/1(In1)  "Delta_rad"
  Gain3/1 -> Sum4/2
  Constant7/1 -> Gain3/1
  Constant3/1 -> Switch/3
  Sum5/1 -> Switch/1
  Unit Delay1/1 -> Sum5/1
  Constant4/1 -> Sum5/2
  Logical Operator1/1 -> Unit Delay2/1, COMM_DONE/1
  Compare To Constant2/1 -> Logical Operator1/1
  Switch/1 -> Unit Delay1/1, Compare To Constant2/1
  Unit Delay2/1 -> Logical Operator1/2
  Sum3/1 -> Compare To Constant/1
  Compare To Constant/1 -> Logical Operator/1
  Abs/1 -> Compare To Constant1/1
  Product/1 -> Gain/1
  Compare To Constant1/1 -> Logical Operator/2
  Constant/1 -> Sum/2
  Logical Operator/1 -> Switch/2, COMM_OK/1
  Bus Selector2/1 -> Sum/1  "<x_m>"
  Bus Selector2/2 -> Sum1/1  "<y_m>"
  Constant1/1 -> Sum1/2
  X/1 -> Bus Selector2/1
  Sum1/1 -> Product1/1, Product1/2
  Gain/1 -> Sum3/1
  Sum/1 -> Product/1, Product/2
  Gain1/1 -> Sum3/2
  Bus Selector2/3 -> Sum4/1  "<tht_rad>"
  Product1/1 -> Gain1/1

== system Bossi_Emanuele_EE460S3D_R99/S3D_Plant/Comm/P3 ==
  X : Inport
  Abs : Abs  SaturateOnIntegerOverflow=off
  Bus Selector2 : BusSelector  OutputSignals=x_m,y_m,tht_rad
  Compare To Constant : simulink/Logic and Bit Operations/Compare To Constant  relop=<=  const=1  OutDataTypeStr=boolean
  Compare To Constant1 : simulink/Logic and Bit Operations/Compare To Constant  relop=<=  const=TOLdata(3,Pdx)  OutDataTypeStr=boolean
  Compare To Constant2 : simulink/Logic and Bit Operations/Compare To Constant  relop=>=  const=LVL.Ptime(Pdx)/dt0  OutDataTypeStr=boolean
  Constant : Constant  Value=Pdata(1,Pdx)  SampleTime=dt0
  Constant1 : Constant  Value=Pdata(2,Pdx)  SampleTime=dt0
  Constant3 : Constant  Value=0  SampleTime=dt0
  Constant4 : Constant  SampleTime=dt0
  Constant7 : Constant  Value=Pdata(3,Pdx)  SampleTime=dt0
  DirectionCompensation2 : Subsystem
  Gain : Gain  Gain=1/(TOLdata(1,Pdx)^2)
  Gain1 : Gain  Gain=1/(TOLdata(2,Pdx)^2)
  Gain3 : Gain  Gain=d2r
  Gain4 : Gain  Gain=r2d
  Logical Operator : Logic  AllPortsSameDT=off  OutDataTypeStr=boolean
  Logical Operator1 : Logic  Operator=OR  AllPortsSameDT=off  OutDataTypeStr=boolean
  Product : Product
  Product1 : Product
  Scope : Scope  NumInputPorts=2
      settings: ActiveDisplayYMinimum=-0.125  ActiveDisplayYMaximum=1.125  DataLoggingVariableName=ScopeData2
  Sum : Sum  Inputs=|+-
  Sum1 : Sum  Inputs=|+-
  Sum3 : Sum  Inputs=|++
  Sum4 : Sum  Inputs=|+-
  Sum5 : Sum  Inputs=++|
  Switch : Switch  Criteria=u2 > Threshold  Threshold=.4  SaturateOnIntegerOverflow=off  InputSameDT=off
  Unit Delay1 : UnitDelay  SampleTime=dt0  HasFrameUpgradeWarning=on
  Unit Delay2 : UnitDelay  SampleTime=dt0  HasFrameUpgradeWarning=on
  COMM_OK : Outport
  COMM_DONE : Outport  Port=2
  wires:
  Gain4/1 -> Abs/1
  DirectionCompensation2/1(Out1) -> Gain4/1
  Sum4/1 -> DirectionCompensation2/1(In1)  "Delta_rad"
  Gain3/1 -> Sum4/2
  Constant7/1 -> Gain3/1
  Constant3/1 -> Switch/3
  Sum5/1 -> Switch/1
  Unit Delay1/1 -> Sum5/1
  Constant4/1 -> Sum5/2
  Logical Operator1/1 -> Unit Delay2/1, COMM_DONE/1
  Compare To Constant2/1 -> Logical Operator1/1
  Switch/1 -> Unit Delay1/1, Compare To Constant2/1
  Unit Delay2/1 -> Logical Operator1/2
  Sum3/1 -> Compare To Constant/1
  Compare To Constant/1 -> Scope/1, Logical Operator/1
  Abs/1 -> Compare To Constant1/1
  Product/1 -> Gain/1
  Compare To Constant1/1 -> Scope/2, Logical Operator/2
  Constant/1 -> Sum/2
  Logical Operator/1 -> Switch/2, COMM_OK/1
  Bus Selector2/1 -> Sum/1  "<x_m>"
  Bus Selector2/2 -> Sum1/1  "<y_m>"
  Constant1/1 -> Sum1/2
  X/1 -> Bus Selector2/1
  Sum1/1 -> Product1/1, Product1/2
  Gain/1 -> Sum3/1
  Sum/1 -> Product/1, Product/2
  Gain1/1 -> Sum3/2
  Bus Selector2/3 -> Sum4/1  "<tht_rad>"
  Product1/1 -> Gain1/1

== system Bossi_Emanuele_EE460S3D_R99/S3D_Plant/Comm/P4 ==
  X : Inport
  Abs : Abs  SaturateOnIntegerOverflow=off
  Bus Selector2 : BusSelector  OutputSignals=x_m,y_m,tht_rad
  Compare To Constant : simulink/Logic and Bit Operations/Compare To Constant  relop=<=  const=1  OutDataTypeStr=boolean
  Compare To Constant1 : simulink/Logic and Bit Operations/Compare To Constant  relop=<=  const=TOLdata(3,Pdx)  OutDataTypeStr=boolean
  Compare To Constant2 : simulink/Logic and Bit Operations/Compare To Constant  relop=>=  const=LVL.Ptime(Pdx)/dt0  OutDataTypeStr=boolean
  Constant : Constant  Value=Pdata(1,Pdx)  SampleTime=dt0
  Constant1 : Constant  Value=Pdata(2,Pdx)  SampleTime=dt0
  Constant3 : Constant  Value=0  SampleTime=dt0
  Constant4 : Constant  SampleTime=dt0
  Constant7 : Constant  Value=Pdata(3,Pdx)  SampleTime=dt0
  DirectionCompensation2 : Subsystem
  Gain : Gain  Gain=1/(TOLdata(1,Pdx)^2)
  Gain1 : Gain  Gain=1/(TOLdata(2,Pdx)^2)
  Gain3 : Gain  Gain=d2r
  Gain4 : Gain  Gain=r2d
  Logical Operator : Logic  AllPortsSameDT=off  OutDataTypeStr=boolean
  Logical Operator1 : Logic  Operator=OR  AllPortsSameDT=off  OutDataTypeStr=boolean
  Product : Product
  Product1 : Product
  Sum : Sum  Inputs=|+-
  Sum1 : Sum  Inputs=|+-
  Sum3 : Sum  Inputs=|++
  Sum4 : Sum  Inputs=|+-
  Sum5 : Sum  Inputs=++|
  Switch : Switch  Criteria=u2 > Threshold  Threshold=.4  SaturateOnIntegerOverflow=off  InputSameDT=off
  Unit Delay1 : UnitDelay  SampleTime=dt0  HasFrameUpgradeWarning=on
  Unit Delay2 : UnitDelay  SampleTime=dt0  HasFrameUpgradeWarning=on
  COMM_OK : Outport
  COMM_DONE : Outport  Port=2
  wires:
  Gain4/1 -> Abs/1
  DirectionCompensation2/1(Out1) -> Gain4/1
  Sum4/1 -> DirectionCompensation2/1(In1)  "Delta_rad"
  Gain3/1 -> Sum4/2
  Constant7/1 -> Gain3/1
  Constant3/1 -> Switch/3
  Sum5/1 -> Switch/1
  Unit Delay1/1 -> Sum5/1
  Constant4/1 -> Sum5/2
  Logical Operator1/1 -> Unit Delay2/1, COMM_DONE/1
  Compare To Constant2/1 -> Logical Operator1/1
  Switch/1 -> Unit Delay1/1, Compare To Constant2/1
  Unit Delay2/1 -> Logical Operator1/2
  Sum3/1 -> Compare To Constant/1
  Compare To Constant/1 -> Logical Operator/1
  Abs/1 -> Compare To Constant1/1
  Product/1 -> Gain/1
  Compare To Constant1/1 -> Logical Operator/2
  Constant/1 -> Sum/2
  Logical Operator/1 -> Switch/2, COMM_OK/1
  Bus Selector2/1 -> Sum/1  "<x_m>"
  Bus Selector2/2 -> Sum1/1  "<y_m>"
  Constant1/1 -> Sum1/2
  X/1 -> Bus Selector2/1
  Sum1/1 -> Product1/1, Product1/2
  Gain/1 -> Sum3/1
  Sum/1 -> Product/1, Product/2
  Gain1/1 -> Sum3/2
  Bus Selector2/3 -> Sum4/1  "<tht_rad>"
  Product1/1 -> Gain1/1

== system Bossi_Emanuele_EE460S3D_R99/S3D_Plant/GetAccel/GetFxb ==
  U : Inport
  Bus Selector : BusSelector  OutputSignals=U1,U2,U3,U4
  Sum : Sum  Inputs=|++
  Sum1 : Sum  Inputs=|++
  Sum2 : Sum  Inputs=|+-
  Fxb : Outport
  wires:
  Bus Selector/3 -> Sum1/1  "<U3>"
  Sum2/1 -> Fxb/1  "Fxb_N"
  Bus Selector/1 -> Sum/1  "<U1>"
  Bus Selector/2 -> Sum/2  "<U2>"
  Sum1/1 -> Sum2/2
  Bus Selector/4 -> Sum1/2  "<U4>"
  Sum/1 -> Sum2/1
  U/1 -> Bus Selector/1

== system Bossi_Emanuele_EE460S3D_R99/S3D_Plant/GetAccel/GetFyb ==
  U : Inport
  Bus Selector : BusSelector  OutputSignals=U5,U8,U6,U7
  Sum3 : Sum  Inputs=|++
  Sum4 : Sum  Inputs=|++
  Sum5 : Sum  Inputs=|-+
  Fyb : Outport
  wires:
  U/1 -> Bus Selector/1
  Bus Selector/4 -> Sum4/2  "<U7>"
  Bus Selector/2 -> Sum3/2  "<U8>"
  Sum3/1 -> Sum5/1
  Sum4/1 -> Sum5/2
  Bus Selector/3 -> Sum4/1  "<U6>"
  Bus Selector/1 -> Sum3/1  "<U5>"
  Sum5/1 -> Fyb/1  "Fyb_N"

== system Bossi_Emanuele_EE460S3D_R99/S3D_Plant/GetAccel/GetMz ==
  U : Inport
  MP : Inport  Port=2
  Bus Selector : BusSelector  OutputSignals=U1,U2,U3,U4,U5,U6,U7,U8  OutputAsBus=on
  Bus Selector3 : BusSelector  OutputSignals=Ycg_m
  Bus Selector4 : BusSelector  OutputSignals=Xcg_m
  Bus to Vector : BusToVector
  Constant1 : Constant  Value=[-1 1 -1 1]  SampleTime=dt0
  Constant2 : Constant  Value=[1 1 -1 -1]  SampleTime=dt0
  Constant3 : Constant  Value=[3 -3 3 -3]  SampleTime=dt0
  Constant4 : Constant  Value=[1 -1 -1 1]  SampleTime=dt0
  Dot Product3 : DotProduct  OutDataTypeStr=Inherit: Inherit via internal rule
  Mux : Mux  Inputs=2
  Product2 : Product
  Product3 : Product
  Sum7 : Sum  Inputs=|++
  Sum8 : Sum  Inputs=|++
  Mzb : Outport
  wires:
  Dot Product3/1 -> Mzb/1  "Mzb_Nm"
  Mux/1 -> Dot Product3/2
  Bus to Vector/1 -> Dot Product3/1
  Bus Selector/1 -> Bus to Vector/1
  Sum8/1 -> Mux/2
  Sum7/1 -> Mux/1
  Product3/1 -> Sum8/2
  Constant3/1 -> Sum8/1
  Bus Selector4/1 -> Product3/2  "<Xcg_m>"
  Constant4/1 -> Product3/1
  MP/1 -> Bus Selector3/1, Bus Selector4/1
  Product2/1 -> Sum7/2
  Constant1/1 -> Sum7/1
  Bus Selector3/1 -> Product2/2  "<Ycg_m>"
  Constant2/1 -> Product2/1
  U/1 -> Bus Selector/1

== system Bossi_Emanuele_EE460S3D_R99/S3D_Plant/GetAccel/InertialAccel ==
  FM : Inport
  MP : Inport  Port=2
  X : Inport  Port=3
  Bus Creator : BusCreator  Inputs=3
  Bus Selector : BusSelector  OutputSignals=Fxb_N,Fyb_N
  Bus Selector{1,3,5,7} (4 alike) : BusSelector  OutputSignals=tht_rad
  Bus Selector2 : BusSelector  OutputSignals=M_kg
  Bus Selector4 : BusSelector  OutputSignals=Fxb_N,Fyb_N
  Bus Selector6 : BusSelector  OutputSignals=M_kg
  Bus Selector8 : BusSelector  OutputSignals=Mzb_Nm
  Bus Selector9 : BusSelector  OutputSignals=J_kgm2
  Product{1..2,4..5} (4 alike) : Product
  Product3 : Product  Inputs=*/
  Product6 : Product  Inputs=*/
  Product7 : Product  Inputs=*/
  Sum1 : Sum  Inputs=|+-
  Sum2 : Sum  Inputs=|++
  Trigonometric Function : Trigonometry
  Trigonometric Function1 : Trigonometry  Operator=cos
  Trigonometric Function2 : Trigonometry  Operator=cos
  Trigonometric Function3 : Trigonometry
  ACCEL : Outport
  wires:
  Bus Creator/1 -> ACCEL/1  "ACCEL"
  Product7/1 -> Bus Creator/3  "thtddt_rps2"
  Product3/1 -> Bus Creator/1  "xddt_mps2"
  Product6/1 -> Bus Creator/2  "yddt_mps2"
  Bus Selector6/1 -> Product6/2  "<M_kg>"
  FM/1 -> Bus Selector/1, Bus Selector4/1, Bus Selector8/1
  Bus Selector9/1 -> Product7/2  "<J_kgm2>"
  Bus Selector8/1 -> Product7/1  "<Mzb_Nm>"
  Bus Selector7/1 -> Trigonometric Function2/1  "<tht_rad>"
  Sum2/1 -> Product6/1
  Bus Selector5/1 -> Trigonometric Function3/1  "<tht_rad>"
  Product4/1 -> Sum2/1
  Bus Selector4/1 -> Product4/2  "<Fxb_N>"
  Bus Selector4/2 -> Product5/1  "<Fyb_N>"
  Trigonometric Function2/1 -> Product5/2
  X/1 -> Bus Selector3/1, Bus Selector5/1, Bus Selector7/1, Bus Selector1/1
  Product5/1 -> Sum2/2
  Trigonometric Function3/1 -> Product4/1
  Trigonometric Function1/1 -> Product1/1
  Product2/1 -> Sum1/2
  Trigonometric Function/1 -> Product2/2
  Bus Selector/2 -> Product2/1  "<Fyb_N>"
  Bus Selector/1 -> Product1/2  "<Fxb_N>"
  MP/1 -> Bus Selector9/1, Bus Selector6/1, Bus Selector2/1
  Product1/1 -> Sum1/1
  Bus Selector1/1 -> Trigonometric Function1/1  "<tht_rad>"
  Bus Selector2/1 -> Product3/2  "<M_kg>"
  Sum1/1 -> Product3/1
  Bus Selector3/1 -> Trigonometric Function/1  "<tht_rad>"

== system Bossi_Emanuele_EE460S3D_R99/S3D_Plant/Integrate/ABM_INT1 ==
  DX : Inport
  Gain : Gain  Gain=23
  Gain1 : Gain  Gain=16
  Gain2 : Gain  Gain=5
  Product : Product  RndMeth=Zero
  Sum : Sum  Inputs=+-+
  Sum2 : Sum  Inputs=++|
  Unit Delay : UnitDelay  SampleTime=dt0  HasFrameUpgradeWarning=on
  Unit Delay1 : UnitDelay  SampleTime=dt0  HasFrameUpgradeWarning=on
  Unit Delay2 : UnitDelay  SampleTime=dt0  HasFrameUpgradeWarning=on
  dt/12 : Constant  Value=dt0/12  SampleTime=dt0
  X : Outport
  wires:
  Gain/1 -> Sum/1
  Gain2/1 -> Sum/3
  Gain1/1 -> Sum/2
  Sum/1 -> Product/2
  DX/1 -> Gain/1, Unit Delay1/1
  Unit Delay/1 -> X/1, Sum2/1  "X"
  Product/1 -> Sum2/2
  Unit Delay1/1 -> Gain1/1, Unit Delay2/1
  Unit Delay2/1 -> Gain2/1
  dt/12/1 -> Product/1
  Sum2/1 -> Unit Delay/1

== system Bossi_Emanuele_EE460S3D_R99/S3D_Plant/Integrate/CentroidData ==
  MP : Inport
  XCG : Inport  Port=2
  Bus Creator : BusCreator  Inputs=9
  Bus Selector4 : BusSelector  OutputSignals=tht_rad,thtdt_rps,thtddt_rps2
  FindCentroid : Subsystem
  FindCentroidAccel : Subsystem
  FindCentroidRates : Subsystem
  XCentroid : Outport
  wires:
  Bus Selector4/3 -> Bus Creator/9  "<thtddt_rps2>"
  Bus Selector4/2 -> Bus Creator/8  "<thtdt_rps>"
  Bus Selector4/1 -> Bus Creator/7  "<tht_rad>"
  FindCentroidAccel/1(Xddtcentroid) -> Bus Creator/5
  FindCentroidAccel/2(Yddtcentroid) -> Bus Creator/6
  FindCentroidRates/1(Xdtcentroid) -> Bus Creator/3
  FindCentroidRates/2(Ydtcentroid) -> Bus Creator/4
  FindCentroid/2(Ycentroid) -> Bus Creator/2
  FindCentroid/1(Xcentroid) -> Bus Creator/1
  XCG/1 -> FindCentroid/2(XCG), FindCentroidRates/2(XCG), FindCentroidAccel/2(XCG), Bus Selector4/1
  MP/1 -> FindCentroid/1(MP), FindCentroidRates/1(MP), FindCentroidAccel/1(MP)
  Bus Creator/1 -> XCentroid/1  "XCentroid"

== system Bossi_Emanuele_EE460S3D_R99/S3D_Plant/MassProperties/GetCGnJ ==
  MfuelVector : Inport
  M_kg : Inport  Port=2
  Constant1 : Constant  Value=[L13 L24 L13 L24].^2  SampleTime=dt0
  Constant2 : Constant  Value=[-3 -2 3 2]  SampleTime=dt0
  Constant3 : Constant  Value=[1 -1.5 -1 1.5]  SampleTime=dt0
  Constant4 : Constant  Value=[17 8 17 8]./12  SampleTime=dt0
  Constant5 : Constant  Value=Jbase+JC0  SampleTime=dt0
  Dot Product{,1..3} (4 alike) : DotProduct  OutDataTypeStr=Inherit: Inherit via internal rule
  Subsystem : Subsystem
  Sum1 : Sum  Inputs=+++
  Sum2 : Sum  Inputs=|++
  Xcg : Outport
  Ycg : Outport  Port=2
  J : Outport  Port=3
  wires:
  MfuelVector/1 -> Dot Product1/2, Dot Product/2, Dot Product3/2, Dot Product2/2
  Sum2/1 -> J/1  "J_kgm2"
  Subsystem/1(Jpat) -> Sum2/2
  Sum1/1 -> Sum2/1
  Constant5/1 -> Sum1/1
  Dot Product3/1 -> Sum1/2
  Dot Product2/1 -> Sum1/3
  Constant1/1 -> Dot Product2/1
  Constant4/1 -> Dot Product3/1
  Subsystem/3(Ycg) -> Ycg/1
  Subsystem/2(Xcg) -> Xcg/1
  M_kg/1 -> Subsystem/3(M_kg)
  Dot Product1/1 -> Subsystem/2(Ymom)  "Ymom"
  Dot Product/1 -> Subsystem/1(Xmom)  "Xmom"
  Constant3/1 -> Dot Product1/1
  Constant2/1 -> Dot Product/1

== system Bossi_Emanuele_EE460S3D_R99/S3D_Plant/OutputDataProcessing/MakePlot ==
  U : Inport
  Sensors : Inport  Port=2
  MP : Inport  Port=3
  x : Inport  Port=4
  COMM : Inport  Port=5
  Bus Selector : BusSelector  OutputSignals=x_m,y_m,tht_rad  OutputAsBus=on
  Bus Selector1 : BusSelector  OutputSignals=U1,U2,U3,U4,U5,U6,U7,U8  OutputAsBus=on
  Bus Selector2 : BusSelector  OutputSignals=MfuelVector
  Bus Selector3 : BusSelector  OutputSignals=P1OK,P1Done,P2OK,P2Done,P3OK,P3Done,P4OK,P4Done  OutputAsBus=on
  Bus Selector4 : BusSelector  OutputSignals=U1fail,U2fail,U3fail,U4fail,U5fail,U6fail,U7fail,U8fail  OutputAsBus=on
  Bus Selector5 : BusSelector  OutputSignals=S1fail,S2fail,S3fail,S4fail,S5fail,S6fail,S7fail,S8fail,S9fail  OutputAsBus=on
  Bus to Vector{,1..4} (5 alike) : BusToVector
  Constant : Constant  Value=PTvec  SampleTime=dt0
  Data Type Conversion : DataTypeConversion  OutDataTypeStr=double  SaturateOnIntegerOverflow=off  RndMeth=Floor
  Data Type Conversion1 : DataTypeConversion  OutDataTypeStr=double  SaturateOnIntegerOverflow=off  RndMeth=Floor
  Data Type Conversion2 : DataTypeConversion  OutDataTypeStr=double  SaturateOnIntegerOverflow=off  RndMeth=Floor
  Digital Clock : DigitalClock  SampleTime=dt0
  Gain1 : Gain  Gain=.1
  Gain2 : Gain  Gain=.01
  MakePlot : Subsystem
  Mux : Mux  Inputs=8
  Signal Specification : SignalSpecification  Dimensions=[3]
  Signal Specification1 : SignalSpecification  Dimensions=[8]
  To Workspace : ToWorkspace  VariableName=PlotInput  SampleTime=dt0
      settings: MaxDataPoints=1
  wires:
  Data Type Conversion/1 -> Mux/5
  Bus to Vector2/1 -> Data Type Conversion/1
  Bus Selector3/1 -> Bus to Vector2/1
  COMM/1 -> Bus Selector3/1
  Signal Specification1/1 -> Gain2/1
  Constant/1 -> Mux/4
  Gain1/1 -> Mux/3
  Signal Specification/1 -> Bus to Vector/1
  Bus Selector2/1 -> Gain1/1  "<MfuelVector>"
  MP/1 -> Bus Selector2/1
  Bus to Vector1/1 -> Signal Specification1/1
  Bus Selector1/1 -> Bus to Vector1/1
  U/1 -> Bus Selector4/1, Bus Selector1/1
  Bus to Vector/1 -> Mux/1
  Bus Selector/1 -> Signal Specification/1
  Gain2/1 -> Mux/2
  x/1 -> Bus Selector/1
  Mux/1 -> MakePlot/1(PlotData), To Workspace/1  "PlotData"
  Digital Clock/1 -> Mux/6
  Bus Selector4/1 -> Bus to Vector3/1
  Bus to Vector3/1 -> Data Type Conversion1/1
  Data Type Conversion1/1 -> Mux/7
  Bus to Vector4/1 -> Data Type Conversion2/1
  Bus Selector5/1 -> Bus to Vector4/1
  Sensors/1 -> Bus Selector5/1
  Data Type Conversion2/1 -> Mux/8

== system Bossi_Emanuele_EE460S3D_R99/S3D_Plant/Sensors/CASE1 ==
  X : Inport
  Action Port : ActionPort  ActionPortLabel=case [ 1 ]:
  Constant2 : Constant  Value=SSF  SampleTime=dt0
  Gain : Gain
  Mux{,1..3} (4 alike) : Mux  Inputs=3
  Product : Product
  THTaccel : Subsystem
  THTpos1 : Subsystem
  THTvel : Subsystem
  Xaccel : Subsystem
  Xpos1 : Subsystem
  Xvel : Subsystem
  Yaccel : Subsystem
  Ypos1 : Subsystem
  Yvel : Subsystem
  Out1 : Outport
  wires:
  Constant2/1 -> Product/2
  Product/1 -> Gain/1
  Mux3/1 -> Product/1
  Gain/1 -> Out1/1
  THTaccel/1(thtddt1) -> Mux2/3
  THTvel/1(thtdt1) -> Mux2/2
  THTpos1/1(tht1) -> Mux2/1
  Mux2/1 -> Mux3/3
  Yaccel/1(yddt1) -> Mux1/3
  Yvel/1(ydt1) -> Mux1/2
  Ypos1/1(y1) -> Mux1/1
  Mux1/1 -> Mux3/2
  Mux/1 -> Mux3/1
  Xaccel/1(xddt1) -> Mux/3
  Xpos1/1(x1) -> Mux/1
  Xvel/1(xdt1) -> Mux/2
  X/1 -> Xpos1/1(X), Xvel/1(X), Xaccel/1(X), Ypos1/1(X), Yvel/1(X), Yaccel/1(X), THTpos1/1(X), THTvel/1(X), THTaccel/1(X)

== system Bossi_Emanuele_EE460S3D_R99/S3D_Plant/Sensors/CASE2 ==
  X : Inport
  Action Port : ActionPort  ActionPortLabel=case [ 2 ]:
  Constant2 : Constant  Value=SSF([1 1 2 4 4 5 7 7 8])  SampleTime=dt0
  Gain : Gain
  Mux{,1..3} (4 alike) : Mux  Inputs=3
  Product : Product
  THTpos1 : Subsystem
  THTpos2 : Subsystem
  THTvel : Subsystem
  Xpos1 : Subsystem
  Xpos2 : Subsystem
  Xvel : Subsystem
  Ypos1 : Subsystem
  Ypos2 : Subsystem
  Yvel : Subsystem
  Out1 : Outport
  wires:
  Constant2/1 -> Product/2
  Product/1 -> Gain/1
  Mux3/1 -> Product/1
  Gain/1 -> Out1/1
  X/1 -> THTvel/1(X), THTpos2/1(X), THTpos1/1(X), Yvel/1(X), Ypos2/1(X), Ypos1/1(X), Xvel/1(X), Xpos2/1(X), Xpos1/1(X)
  Xpos2/1(x1) -> Mux/2
  Xpos1/1(x1) -> Mux/1
  Xvel/1(xdt1) -> Mux/3
  Mux/1 -> Mux3/1
  Mux1/1 -> Mux3/2
  Ypos1/1(y1) -> Mux1/1
  Ypos2/1(y1) -> Mux1/2
  Yvel/1(ydt1) -> Mux1/3
  Mux2/1 -> Mux3/3
  THTpos1/1(tht1) -> Mux2/1
  THTpos2/1(tht1) -> Mux2/2
  THTvel/1(thtdt1) -> Mux2/3

== system Bossi_Emanuele_EE460S3D_R99/S3D_Plant/Sensors/CASE3 ==
  X : Inport
  Action Port : ActionPort  ActionPortLabel=default:
  Constant2 : Constant  Value=SSF([1 1 1 4 4 4 7 7 7])  SampleTime=dt0
  Gain : Gain
  Mux{,1..3} (4 alike) : Mux  Inputs=3
  Product : Product
  THTpos1 : Subsystem
  THTpos2 : Subsystem
  THTpos3 : Subsystem
  Xpos1 : Subsystem
  Xpos2 : Subsystem
  Xpos3 : Subsystem
  Ypos1 : Subsystem
  Ypos2 : Subsystem
  Ypos3 : Subsystem
  Out1 : Outport
  wires:
  Constant2/1 -> Product/2
  Product/1 -> Gain/1
  Mux3/1 -> Product/1
  Gain/1 -> Out1/1
  THTpos3/1(tht1) -> Mux2/3
  THTpos2/1(tht1) -> Mux2/2
  THTpos1/1(tht1) -> Mux2/1
  Mux2/1 -> Mux3/3
  Ypos3/1(y1) -> Mux1/3
  Ypos2/1(y1) -> Mux1/2
  Ypos1/1(y1) -> Mux1/1
  Mux1/1 -> Mux3/2
  Mux/1 -> Mux3/1
  Xpos3/1(xddt1) -> Mux/3
  Xpos1/1(x1) -> Mux/1
  Xpos2/1(xdt1) -> Mux/2
  X/1 -> Xpos1/1(X), Ypos1/1(X), THTpos1/1(X), THTpos2/1(X), THTpos3/1(X), Ypos3/1(X), Ypos2/1(X), Xpos3/1(X), Xpos2/1(X)
